simulink model "series_3"  (R2025b)
settings: Solver=VariableStepAuto  StartTime=0.0  StopTime=3600  RelTol=1e-3  AbsTol=1e-3
libraries: customization_lib x13, nesl_utility x1
settings Model: Creator=degoede  LastModifiedBy=degoede
settings SimscapeCC: SimscapeLogType=all  SimscapeLogSimulationStatistics=on  SimscapeLogOpenViewer=on

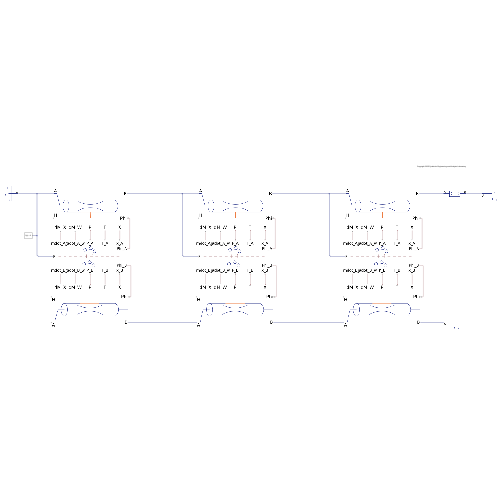
[thumbnail: Simulink's stored preview of the top-level diagram]
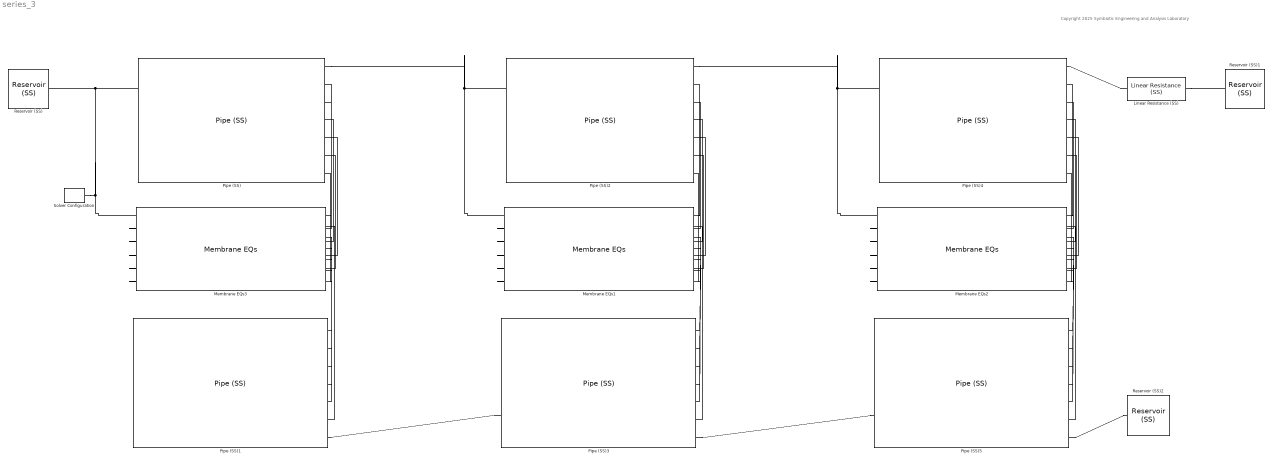
== system series_3 ==
  note: Copyright 2025 Symbiotic Engineering and Analysis Laboratory
  Linear Resistance (SS) : customization_lib/solution/elements/Linear Resistance (SS)  R=64230000 Pa*s/m^3  area=0.01 m^2
      settings: SourceProductName=Customization  InternalSimscapePortConfiguration="{\"Bottom\":[],\"Left\":[{\"id\":\"A\",\"label\":\"A\",\"type\":\"customization.solution.solution\"}],\"Right\":[{\"id\":\"B\",\"label\":\"B\",\"type\":\"customization.solution.solution\"}],\"Top\":[]}"
  Membrane EQs1 : customization_lib/membranes/Membrane EQs  A_w=2.57e-12 m^3/(N*s)  B_s=2.30e-8 m/s  A_m=35 m^2
      settings: SourceProductName=Customization  InternalSimscapePortConfiguration="{\"Bottom\":[{\"id\":\"mdot_B_x\",\"label\":\"mdot_B_x\",\"type\":\"output\"},{\"id\":\"mdot_B_w\",\"label\":\"mdot_B_w\",\"type\":\"output\"},{\"id\":\"P_B\",\"label\":\"P_B\",\"type\":\"input\"},{\"id\":\"T_B\",\"label\":\"T_B\",\"type\":\"input\"},{\"id\":\"x_B\",\"label\":\"x_B\",\"type\":\"input\"}],\"Left\":[{\"id\":\"F\",\"label\":\"F\",\"type\":\"customization.solution.solution\"}],\"Right\":[{\"id\":\"Phi_A\",\"label\":\"Phi_A\",\"type\":\"output\"},{\"id\":\"Phi_B\",\"label\":\"Phi_B\",\"type\":\"output\"}],\"Top\":[{\"id\":\"mdot_A_x\",\"label\":\"mdot_A_x\",\"type\":\"output\"},{\"id\":\"mdot_A_w\",\"label\":\"mdot_A_w\",\"type\":\"output\"},{\"id\":\"P_A\",\"label\":\"P_A\",\"type\":\"input\"},{\"id\":\"T_A\",\"label\":\"T_A\",\"type\":\"input\"},{\"id\":\"x_A\",\"label\":\"x_A\",\"type\":\"input\"}]}"
  Membrane EQs2 : customization_lib/membranes/Membrane EQs  A_w=2.57e-12 m^3/(N*s)  B_s=2.30e-8 m/s  A_m=35 m^2
      settings: SourceProductName=Customization  InternalSimscapePortConfiguration="{\"Bottom\":[{\"id\":\"mdot_B_x\",\"label\":\"mdot_B_x\",\"type\":\"output\"},{\"id\":\"mdot_B_w\",\"label\":\"mdot_B_w\",\"type\":\"output\"},{\"id\":\"P_B\",\"label\":\"P_B\",\"type\":\"input\"},{\"id\":\"T_B\",\"label\":\"T_B\",\"type\":\"input\"},{\"id\":\"x_B\",\"label\":\"x_B\",\"type\":\"input\"}],\"Left\":[{\"id\":\"F\",\"label\":\"F\",\"type\":\"customization.solution.solution\"}],\"Right\":[{\"id\":\"Phi_A\",\"label\":\"Phi_A\",\"type\":\"output\"},{\"id\":\"Phi_B\",\"label\":\"Phi_B\",\"type\":\"output\"}],\"Top\":[{\"id\":\"mdot_A_x\",\"label\":\"mdot_A_x\",\"type\":\"output\"},{\"id\":\"mdot_A_w\",\"label\":\"mdot_A_w\",\"type\":\"output\"},{\"id\":\"P_A\",\"label\":\"P_A\",\"type\":\"input\"},{\"id\":\"T_A\",\"label\":\"T_A\",\"type\":\"input\"},{\"id\":\"x_A\",\"label\":\"x_A\",\"type\":\"input\"}]}"
  Membrane EQs3 : customization_lib/membranes/Membrane EQs  A_w=2.57e-12 m^3/(N*s)  B_s=2.30e-8 m/s  A_m=35 m^2
      settings: SourceProductName=Customization  InternalSimscapePortConfiguration="{\"Bottom\":[{\"id\":\"mdot_B_x\",\"label\":\"mdot_B_x\",\"type\":\"output\"},{\"id\":\"mdot_B_w\",\"label\":\"mdot_B_w\",\"type\":\"output\"},{\"id\":\"P_B\",\"label\":\"P_B\",\"type\":\"input\"},{\"id\":\"T_B\",\"label\":\"T_B\",\"type\":\"input\"},{\"id\":\"x_B\",\"label\":\"x_B\",\"type\":\"input\"}],\"Left\":[{\"id\":\"F\",\"label\":\"F\",\"type\":\"customization.solution.solution\"}],\"Right\":[{\"id\":\"Phi_A\",\"label\":\"Phi_A\",\"type\":\"output\"},{\"id\":\"Phi_B\",\"label\":\"Phi_B\",\"type\":\"output\"}],\"Top\":[{\"id\":\"mdot_A_x\",\"label\":\"mdot_A_x\",\"type\":\"output\"},{\"id\":\"mdot_A_w\",\"label\":\"mdot_A_w\",\"type\":\"output\"},{\"id\":\"P_A\",\"label\":\"P_A\",\"type\":\"input\"},{\"id\":\"T_A\",\"label\":\"T_A\",\"type\":\"input\"},{\"id\":\"x_A\",\"label\":\"x_A\",\"type\":\"input\"}]}"
  Pipe (SS) : customization_lib/solution/elements/Pipe (SS)  length=3.33 m  area=1071000 mm^2  Dh=2.125 mm  length_add=0 m  roughness=1.5e-05 m  Re_lam=2000  Re_tur=4000  shape_factor=64  Nu_lam=3.66  dynamic_compressibility=true  inertia=false  p0=7 MPa  T0=293.15 K  x0=50 kg/m^3  mdot0=0 kg/s  m_measure=false  p_measure=true  t_measure=true  x_measure=true
      settings: SourceProductName=Customization  InternalSimscapePortConfiguration="{\"Bottom\":[{\"id\":\"dM_X\",\"label\":\"dM_X\",\"type\":\"input\"},{\"id\":\"dM_W\",\"label\":\"dM_W\",\"type\":\"input\"},{\"id\":\"P\",\"label\":\"P\",\"type\":\"output\"},{\"id\":\"T\",\"label\":\"T\",\"type\":\"output\"},{\"id\":\"X\",\"label\":\"X\",\"type\":\"output\"}],\"Left\":[{\"id\":\"A\",\"label\":\"A\",\"type\":\"customization.solution.solution\"},{\"id\":\"H\",\"label\":\"H\",\"type\":\"foundation.thermal.thermal\"}],\"Right\":[{\"id\":\"B\",\"label\":\"B\",\"type\":\"customization.solution.solution\"},{\"id\":\"Phi\",\"label\":\"Phi\",\"type\":\"input\"}],\"Top\":[]}"
  Pipe (SS)1 : customization_lib/solution/elements/Pipe (SS)  length=10 m  area=490.873852123405 mm^2  Dh=25 mm  length_add=0 m  roughness=1.5e-05 m  Re_lam=2000  Re_tur=4000  shape_factor=64  Nu_lam=3.66  dynamic_compressibility=true  inertia=false  p0=0.101 MPa  T0=293.15 K  x0=0 kg/m^3  mdot0=0 kg/s  m_measure=false  p_measure=true  t_measure=true  x_measure=true
      settings: SourceProductName=Customization  InternalSimscapePortConfiguration="{\"Bottom\":[{\"id\":\"dM_X\",\"label\":\"dM_X\",\"type\":\"input\"},{\"id\":\"dM_W\",\"label\":\"dM_W\",\"type\":\"input\"},{\"id\":\"P\",\"label\":\"P\",\"type\":\"output\"},{\"id\":\"T\",\"label\":\"T\",\"type\":\"output\"},{\"id\":\"X\",\"label\":\"X\",\"type\":\"output\"}],\"Left\":[{\"id\":\"A\",\"label\":\"A\",\"type\":\"customization.solution.solution\"},{\"id\":\"H\",\"label\":\"H\",\"type\":\"foundation.thermal.thermal\"}],\"Right\":[{\"id\":\"B\",\"label\":\"B\",\"type\":\"customization.solution.solution\"},{\"id\":\"Phi\",\"label\":\"Phi\",\"type\":\"input\"}],\"Top\":[]}"
  Pipe (SS)2 : customization_lib/solution/elements/Pipe (SS)  length=3.33 m  area=1071000 mm^2  Dh=2.125 mm  length_add=0 m  roughness=1.5e-05 m  Re_lam=2000  Re_tur=4000  shape_factor=64  Nu_lam=3.66  dynamic_compressibility=true  inertia=false  p0=7 MPa  T0=293.15 K  x0=50 kg/m^3  mdot0=0 kg/s  m_measure=false  p_measure=true  t_measure=true  x_measure=true
      settings: SourceProductName=Customization  InternalSimscapePortConfiguration="{\"Bottom\":[{\"id\":\"dM_X\",\"label\":\"dM_X\",\"type\":\"input\"},{\"id\":\"dM_W\",\"label\":\"dM_W\",\"type\":\"input\"},{\"id\":\"P\",\"label\":\"P\",\"type\":\"output\"},{\"id\":\"T\",\"label\":\"T\",\"type\":\"output\"},{\"id\":\"X\",\"label\":\"X\",\"type\":\"output\"}],\"Left\":[{\"id\":\"A\",\"label\":\"A\",\"type\":\"customization.solution.solution\"},{\"id\":\"H\",\"label\":\"H\",\"type\":\"foundation.thermal.thermal\"}],\"Right\":[{\"id\":\"B\",\"label\":\"B\",\"type\":\"customization.solution.solution\"},{\"id\":\"Phi\",\"label\":\"Phi\",\"type\":\"input\"}],\"Top\":[]}"
  Pipe (SS)3 : customization_lib/solution/elements/Pipe (SS)  length=10 m  area=490.873852123405 mm^2  Dh=25 mm  length_add=0 m  roughness=1.5e-05 m  Re_lam=2000  Re_tur=4000  shape_factor=64  Nu_lam=3.66  dynamic_compressibility=true  inertia=false  p0=0.101 MPa  T0=293.15 K  x0=0 kg/m^3  mdot0=0 kg/s  m_measure=false  p_measure=true  t_measure=true  x_measure=true
      settings: SourceProductName=Customization  InternalSimscapePortConfiguration="{\"Bottom\":[{\"id\":\"dM_X\",\"label\":\"dM_X\",\"type\":\"input\"},{\"id\":\"dM_W\",\"label\":\"dM_W\",\"type\":\"input\"},{\"id\":\"P\",\"label\":\"P\",\"type\":\"output\"},{\"id\":\"T\",\"label\":\"T\",\"type\":\"output\"},{\"id\":\"X\",\"label\":\"X\",\"type\":\"output\"}],\"Left\":[{\"id\":\"A\",\"label\":\"A\",\"type\":\"customization.solution.solution\"},{\"id\":\"H\",\"label\":\"H\",\"type\":\"foundation.thermal.thermal\"}],\"Right\":[{\"id\":\"B\",\"label\":\"B\",\"type\":\"customization.solution.solution\"},{\"id\":\"Phi\",\"label\":\"Phi\",\"type\":\"input\"}],\"Top\":[]}"
  Pipe (SS)4 : customization_lib/solution/elements/Pipe (SS)  length=3.33 m  area=1071000 mm^2  Dh=2.125 mm  length_add=0 m  roughness=1.5e-05 m  Re_lam=2000  Re_tur=4000  shape_factor=64  Nu_lam=3.66  dynamic_compressibility=true  inertia=false  p0=7 MPa  T0=293.15 K  x0=50 kg/m^3  mdot0=0 kg/s  m_measure=false  p_measure=true  t_measure=true  x_measure=true
      settings: SourceProductName=Customization  InternalSimscapePortConfiguration="{\"Bottom\":[{\"id\":\"dM_X\",\"label\":\"dM_X\",\"type\":\"input\"},{\"id\":\"dM_W\",\"label\":\"dM_W\",\"type\":\"input\"},{\"id\":\"P\",\"label\":\"P\",\"type\":\"output\"},{\"id\":\"T\",\"label\":\"T\",\"type\":\"output\"},{\"id\":\"X\",\"label\":\"X\",\"type\":\"output\"}],\"Left\":[{\"id\":\"A\",\"label\":\"A\",\"type\":\"customization.solution.solution\"},{\"id\":\"H\",\"label\":\"H\",\"type\":\"foundation.thermal.thermal\"}],\"Right\":[{\"id\":\"B\",\"label\":\"B\",\"type\":\"customization.solution.solution\"},{\"id\":\"Phi\",\"label\":\"Phi\",\"type\":\"input\"}],\"Top\":[]}"
  Pipe (SS)5 : customization_lib/solution/elements/Pipe (SS)  length=10 m  area=490.873852123405 mm^2  Dh=25 mm  length_add=0 m  roughness=1.5e-05 m  Re_lam=2000  Re_tur=4000  shape_factor=64  Nu_lam=3.66  dynamic_compressibility=true  inertia=false  p0=0.101 MPa  T0=293.15 K  x0=0 kg/m^3  mdot0=0 kg/s  m_measure=false  p_measure=true  t_measure=true  x_measure=true
      settings: SourceProductName=Customization  InternalSimscapePortConfiguration="{\"Bottom\":[{\"id\":\"dM_X\",\"label\":\"dM_X\",\"type\":\"input\"},{\"id\":\"dM_W\",\"label\":\"dM_W\",\"type\":\"input\"},{\"id\":\"P\",\"label\":\"P\",\"type\":\"output\"},{\"id\":\"T\",\"label\":\"T\",\"type\":\"output\"},{\"id\":\"X\",\"label\":\"X\",\"type\":\"output\"}],\"Left\":[{\"id\":\"A\",\"label\":\"A\",\"type\":\"customization.solution.solution\"},{\"id\":\"H\",\"label\":\"H\",\"type\":\"foundation.thermal.thermal\"}],\"Right\":[{\"id\":\"B\",\"label\":\"B\",\"type\":\"customization.solution.solution\"},{\"id\":\"Phi\",\"label\":\"Phi\",\"type\":\"input\"}],\"Top\":[]}"
  Reservoir (SS) : customization_lib/solution/elements/Reservoir (SS)  pressure_spec=foundation.enum.pressure_spec.specified  reservoir_pressure=7 MPa  reservoir_temperature=293.15 K  reservoir_concentration=50 kg/m^3  area=1 cm^2
      settings: SourceProductName=Customization  InternalSimscapePortConfiguration="{\"Bottom\":[],\"Left\":[{\"id\":\"A\",\"label\":\"A\",\"type\":\"customization.solution.solution\"}],\"Right\":[],\"Top\":[]}"
  Reservoir (SS)1 : customization_lib/solution/elements/Reservoir (SS)  pressure_spec=foundation.enum.pressure_spec.atmospheric  reservoir_pressure=0.101325 MPa  reservoir_temperature=293.15 K  reservoir_concentration=50 kg/m^3  area=27 mm^2
      settings: SourceProductName=Customization  InternalSimscapePortConfiguration="{\"Bottom\":[],\"Left\":[{\"id\":\"A\",\"label\":\"A\",\"type\":\"customization.solution.solution\"}],\"Right\":[],\"Top\":[]}"
  Reservoir (SS)2 : customization_lib/solution/elements/Reservoir (SS)  pressure_spec=foundation.enum.pressure_spec.atmospheric  reservoir_pressure=7 MPa  reservoir_temperature=293.15 K  reservoir_concentration=0 kg/m^3  area=1 cm^2
      settings: SourceProductName=Customization  InternalSimscapePortConfiguration="{\"Bottom\":[],\"Left\":[{\"id\":\"A\",\"label\":\"A\",\"type\":\"customization.solution.solution\"}],\"Right\":[],\"Top\":[]}"
  Solver Configuration : nesl_utility/Solver Configuration  PhysicalDomain=network_engine_domain  SubClassName=solver  LeftPortType=input  RightPortType=generic  Tones=[]  Harmonics=[]  SimulateNoise=off  Profile=off  UseLocalSampling=off  EnableSwitchedLinearOptims=on  FrequencyDomain=off  UseCCode=off  RelTol=0.001  AbsTol=0.001  MinStep=1e-09  ToWorkspace=off  RevertToSquareIcSolve=off  NumHomotopyIterations=100  PhasorMode=off  PhasorModeNumHarmonics=1  ConsistencySolver=NEWTON_XTOL_AFTER_FTOL  IndexReductionMethod=DerivativeReplacement  DoDC=off  ResidualTolerance=1e-09  ConsistencyTolSource=GLOBAL  ConsistencyAbsTol=0.001  ConsistencyRelTol=0.001  ConsistencyTolFactor=0.001  UseLocalSolver=off  LocalSolverChoice=NE_BACKWARD_EULER_ADVANCER  ResolveIndetEquations=on  FunctionEvalNumThread=1  LocalSolverSampleTime=0.001  DoFixedCost=off  MaxNonlinIter=3  MaxModeIter=2  ComputeImpulses=off  ImpulseIterations=2  LinearAlgebra=auto  LinearAlgebraNumThread=0  EquationFormulation=NE_TIME_EF  DelaysMemoryBudget=1024  AutomaticFiltering=off  FilteringTimeConstant=0.001  PartitionStorageMethod=AS_NEEDED  PartitionMemoryBudget=1024  PartitionMethod=ROBUST  MultibodyUseLocalSolver=off  MultibodyLocalSolverChoice=ODE1  MultibodyLocalSolverSampleTime=0.001
  connections:
  Solver Configuration/RConn1 -- Membrane EQs3/LConn1 -- Pipe (SS)/LConn1 -- Reservoir (SS)/LConn1
  Linear Resistance (SS)/RConn1 -- Reservoir (SS)1/LConn1
  Pipe (SS)5/RConn1 -- Reservoir (SS)2/LConn1
  Linear Resistance (SS)/LConn1 -- Pipe (SS)4/RConn1
  Membrane EQs3/RConn1 -- Pipe (SS)/RConn2
  Membrane EQs3/LConn6 -- Pipe (SS)/RConn7
  Membrane EQs3/RConn6 -- Pipe (SS)1/RConn6
  Membrane EQs3/LConn2 -- Pipe (SS)/RConn3
  Pipe (SS)3/LConn1 -- Pipe (SS)1/RConn1
  Membrane EQs3/RConn2 -- Pipe (SS)1/RConn2
  Membrane EQs3/LConn3 -- Pipe (SS)/RConn4
  Membrane EQs3/LConn5 -- Pipe (SS)/RConn6
  Membrane EQs3/RConn7 -- Pipe (SS)1/RConn7
  Membrane EQs3/RConn5 -- Pipe (SS)1/RConn5
  Membrane EQs3/RConn4 -- Pipe (SS)1/RConn4
  Membrane EQs3/LConn4 -- Pipe (SS)/RConn5
  Membrane EQs3/RConn3 -- Pipe (SS)1/RConn3
  Pipe (SS)2/LConn1 -- Membrane EQs1/LConn1 -- Pipe (SS)/RConn1
  Membrane EQs1/RConn1 -- Pipe (SS)2/RConn2
  Membrane EQs1/LConn6 -- Pipe (SS)2/RConn7
  Membrane EQs1/RConn6 -- Pipe (SS)3/RConn6
  Membrane EQs1/LConn2 -- Pipe (SS)2/RConn3
  Membrane EQs1/RConn2 -- Pipe (SS)3/RConn2
  Membrane EQs1/LConn3 -- Pipe (SS)2/RConn4
  Membrane EQs1/LConn5 -- Pipe (SS)2/RConn6
  Membrane EQs1/RConn7 -- Pipe (SS)3/RConn7
  Membrane EQs1/RConn5 -- Pipe (SS)3/RConn5
  Membrane EQs1/RConn4 -- Pipe (SS)3/RConn4
  Membrane EQs1/LConn4 -- Pipe (SS)2/RConn5
  Membrane EQs1/RConn3 -- Pipe (SS)3/RConn3
  Pipe (SS)4/LConn1 -- Membrane EQs2/LConn1 -- Pipe (SS)2/RConn1
  Membrane EQs2/RConn1 -- Pipe (SS)4/RConn2
  Membrane EQs2/LConn6 -- Pipe (SS)4/RConn7
  Membrane EQs2/RConn6 -- Pipe (SS)5/RConn6
  Membrane EQs2/LConn2 -- Pipe (SS)4/RConn3
  Membrane EQs2/RConn2 -- Pipe (SS)5/RConn2
  Membrane EQs2/LConn3 -- Pipe (SS)4/RConn4
  Membrane EQs2/LConn5 -- Pipe (SS)4/RConn6
  Membrane EQs2/RConn7 -- Pipe (SS)5/RConn7
  Membrane EQs2/RConn5 -- Pipe (SS)5/RConn5
  Membrane EQs2/RConn4 -- Pipe (SS)5/RConn4
  Membrane EQs2/LConn4 -- Pipe (SS)4/RConn5
  Membrane EQs2/RConn3 -- Pipe (SS)5/RConn3
  Pipe (SS)3/RConn1 -- Pipe (SS)5/LConn1
